simulink model "block_diagram_ode2"  (R2025b)
settings: Solver=ode8  StartTime=0.0  StopTime=10.0  FixedStep=0.01  RelTol=1e-3
settings Model: Creator=MehrSystem  LastModifiedBy=MehrSystem

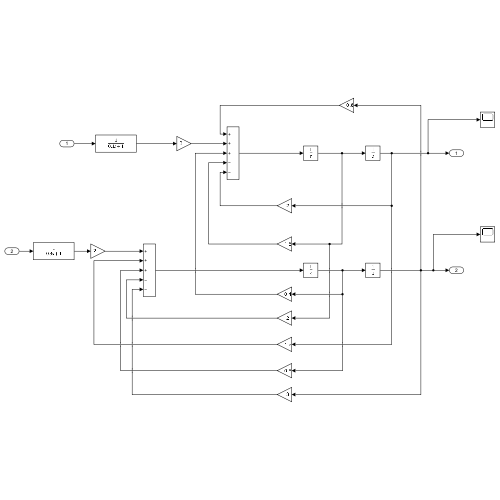
[thumbnail: Simulink's stored preview of the top-level diagram]
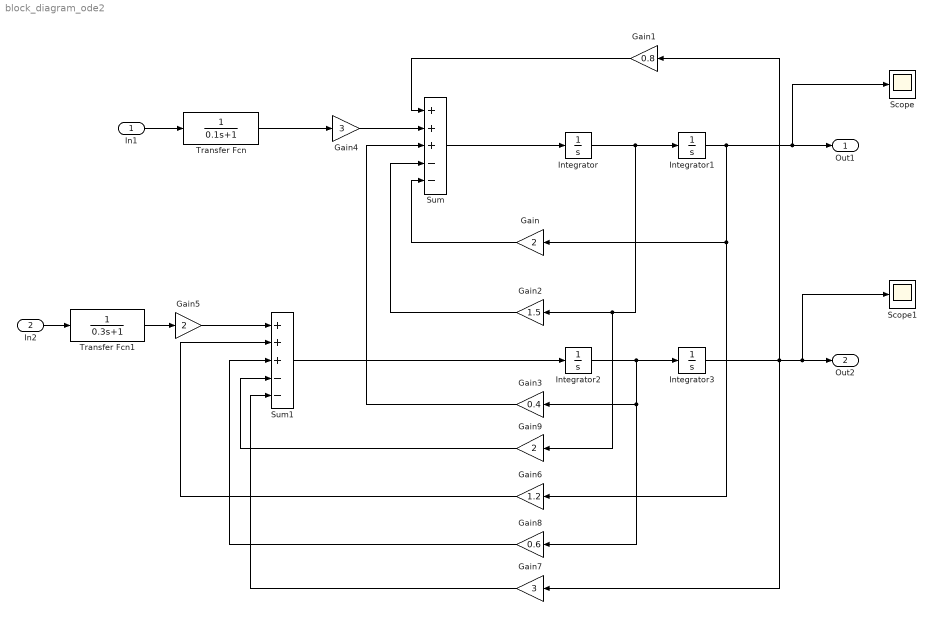
== system block_diagram_ode2 ==
  In1 : Inport
  In2 : Inport  Port=2
  Gain : Gain  Gain=2
  Gain1 : Gain  Gain=0.8
  Gain2 : Gain  Gain=1.5
  Gain3 : Gain  Gain=0.4
  Gain4 : Gain  Gain=3
  Gain5 : Gain  Gain=2
  Gain6 : Gain  Gain=1.2
  Gain7 : Gain  Gain=3
  Gain8 : Gain  Gain=0.6
  Gain9 : Gain  Gain=2
  Integrator{,1..3} (4 alike) : Integrator
  Scope : Scope
  Scope1 : Scope
  Sum : Sum  Inputs=+++--
  Sum1 : Sum  Inputs=+++--
  Transfer Fcn : TransferFcn  Denominator=[0.1 1]
  Transfer Fcn1 : TransferFcn  Denominator=[0.3 1]
  Out1 : Outport
  Out2 : Outport  Port=2
  wires:
  Integrator/1 -> Gain2/1, Gain9/1, Integrator1/1
  Integrator1/1 -> Scope/1, Out1/1, Gain/1, Gain6/1
  Integrator2/1 -> Gain3/1, Gain8/1, Integrator3/1
  Sum/1 -> Integrator/1
  Gain/1 -> Sum/5
  Integrator3/1 -> Gain1/1, Scope1/1, Out2/1, Gain7/1
  Gain1/1 -> Sum/1
  Gain2/1 -> Sum/4
  Gain3/1 -> Sum/3
  In1/1 -> Transfer Fcn/1
  Gain4/1 -> Sum/2
  Sum1/1 -> Integrator2/1
  In2/1 -> Transfer Fcn1/1
  Gain5/1 -> Sum1/1
  Gain6/1 -> Sum1/2
  Gain7/1 -> Sum1/5
  Gain8/1 -> Sum1/3
  Gain9/1 -> Sum1/4
  Transfer Fcn/1 -> Gain4/1
  Transfer Fcn1/1 -> Gain5/1
